simulink model "visualization"  (R2024a)
settings: Solver=VariableStepAuto  StartTime=0.0  StopTime=10.0  RelTol=1e-3
values from neighbouring files (symbols this model uses):
  enable_aircraft_view = 1    [main_chap05_02.m]
libraries: simulink x2
settings Model: Creator=pf  LastModifiedBy=pf

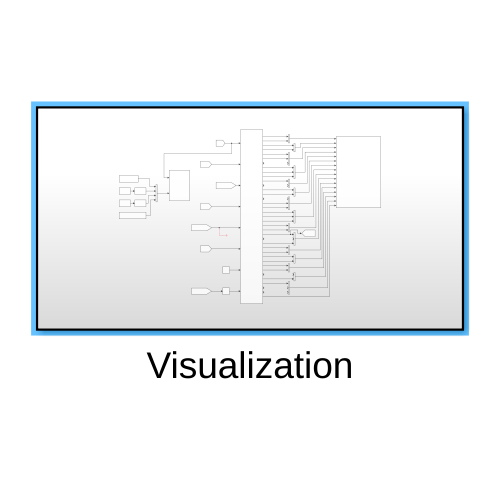
[thumbnail: Simulink's stored preview of the top-level diagram]
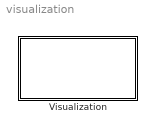
== system visualization ==
  Visualization : Subsystem

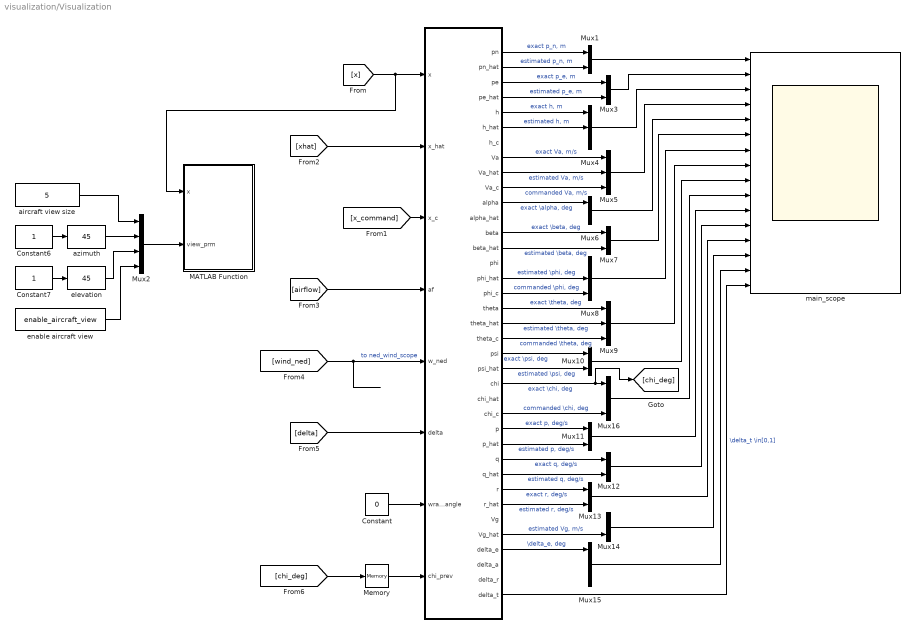
== system visualization/Visualization ==
  " " : MATLAB Function  TreatAsAtomicUnit=on
  Constant : Constant  Value=0
  Constant6 : Constant
  Constant7 : Constant
  MATLAB Function : MATLAB Function  TreatAsAtomicUnit=on
  Memory : Memory
  Mux{1,3,6..7,10..14} (9 alike) : Mux  Inputs=2
  Mux{4..5,8..9,15..16} (6 alike) : Mux  Inputs=3
  Mux2 : Mux
  aircraft view size : Constant  Value=5
  azimuth : simulink/Math Operations/Slider Gain  gain=45  low=-180  high=180
  elevation : simulink/Math Operations/Slider Gain  gain=45  low=-180  high=180
  enable aircraft view : Constant  Value=enable_aircraft_view
  main_scope : Scope  NumInputPorts=16
  wires:
  enable aircraft view/1 -> Mux2/4
  [x] -> MATLAB Function/1(x), " "/1(x)
  azimuth/1 -> Mux2/2
  Constant6/1 -> azimuth/1
  Constant7/1 -> elevation/1
  aircraft view size/1 -> Mux2/1
  Mux2/1 -> MATLAB Function/2(view_prm)
  elevation/1 -> Mux2/3
  [xhat] -> " "/2(x_hat)
  [x_command] -> " "/3(x_c)
  [airflow] -> " "/4(af)
  [wind_ned] -> " "/5(w_ned)  "to ned_wind_scope"
  [delta] -> " "/6(delta)
  Constant/1 -> " "/7(wrap_angle)
  " "/1(pn) -> Mux1/1  "exact p_n, m"
  " "/2(pn_hat) -> Mux1/2  "estimated p_n, m"
  " "/3(pe) -> Mux3/1  "exact p_e, m"
  " "/4(pe_hat) -> Mux3/2  "estimated p_e, m"
  " "/5(h) -> Mux4/1  "exact h, m"
  " "/6(h_hat) -> Mux4/2  "estimated h, m"
  " "/9(Va_hat) -> Mux5/2  "estimated Va, m/s"
  " "/10(Va_c) -> Mux5/3  "commanded Va, m/s"
  " "/8(Va) -> Mux5/1  "exact Va, m/s"
  " "/11(alpha) -> Mux6/1  "exact \\alpha, deg"
  " "/13(beta) -> Mux7/1  "exact \\beta, deg"
  " "/14(beta_hat) -> Mux7/2  "estimated \\beta, deg"
  " "/16(phi_hat) -> Mux8/2  "estimated \\phi, deg"
  " "/17(phi_c) -> Mux8/3  "commanded \\phi, deg"
  " "/19(theta_hat) -> Mux9/2  "estimated \\theta, deg"
  " "/18(theta) -> Mux9/1  "exact \\theta, deg"
  " "/20(theta_c) -> Mux9/3  "commanded \\theta, deg"
  " "/21(psi) -> Mux10/1  "exact \\psi, deg"
  " "/22(psi_hat) -> Mux10/2  "estimated \\psi, deg"
  " "/23(chi) -> [chi_deg], Mux16/1  "exact \\chi, deg"
  " "/25(chi_c) -> Mux16/3  "commanded \\chi, deg"
  " "/27(p_hat) -> Mux11/2  "estimated p, deg/s"
  " "/26(p) -> Mux11/1  "exact p, deg/s"
  " "/28(q) -> Mux12/1  "exact q, deg/s"
  " "/29(q_hat) -> Mux12/2  "estimated q, deg/s"
  " "/30(r) -> Mux13/1  "exact r, deg/s"
  " "/31(r_hat) -> Mux13/2  "estimated r, deg/s"
  " "/33(Vg_hat) -> Mux14/2  "estimated Vg, m/s"
  " "/34(delta_e) -> Mux15/1  "\\delta_e, deg"
  " "/37(delta_t) -> main_scope/16  "\\delta_t \\in[0,1]"
  Mux15/1 -> main_scope/15
  Mux14/1 -> main_scope/14
  Mux13/1 -> main_scope/13
  Mux12/1 -> main_scope/12
  Mux11/1 -> main_scope/11
  Mux9/1 -> main_scope/8
  Mux8/1 -> main_scope/7
  Mux7/1 -> main_scope/6
  Mux6/1 -> main_scope/5
  Mux5/1 -> main_scope/4
  Mux4/1 -> main_scope/3
  Mux3/1 -> main_scope/2
  Mux1/1 -> main_scope/1
  Mux10/1 -> main_scope/9
  Mux16/1 -> main_scope/10
  Memory/1 -> " "/8(chi_prev)
  [chi_deg] -> Memory/1

== matlab function visualization/Visualization/MATLAB Function ==
  data: x input; view_prm input
function draw_aircraft_fcn(x,view_prm)
    draw_aircraft(x,view_prm);
end

== matlab function visualization/Visualization/  ==
  data: x input; x_hat input; x_c input; af input; w_ned input; delta input; wrap_angle input; chi_prev input; pn output; pn_hat output; pe output; pe_hat output; h output; h_hat output; h_c output; Va output; Va_hat output; Va_c output; alpha output; alpha_hat output; beta output; beta_hat output; phi output; phi_hat output; phi_c output; theta output; theta_hat output; theta_c output; psi output; psi_hat output; chi output; chi_hat output; chi_c output; p output; p_hat output; q output; q_hat output; r output; r_hat output; Vg output; Vg_hat output; delta_e output; delta_a output; delta_r output; delta_t output
function [  pn, pn_hat, ...
            pe, pe_hat, ...
            h, h_hat, h_c, ...
            Va, Va_hat, Va_c, ...
            alpha, alpha_hat, ...
            beta, beta_hat, ...
            phi, phi_hat, phi_c, ...
            theta, theta_hat, theta_c, ...
            psi, psi_hat, ...
            chi, chi_hat, chi_c, ...
            p, p_hat, ...
            q, q_hat, ...
            r, r_hat, ...
            Vg, Vg_hat, ...
            delta_e,delta_a,delta_r,delta_t] = ...
            fcn(x,x_hat,x_c,af,w_ned,delta,wrap_angle,chi_prev)

    [  pn, pn_hat, ...
            pe, pe_hat, ...
            h, h_hat, h_c, ...
            Va, Va_hat, Va_c, ...
            alpha, alpha_hat, ...
            beta, beta_hat, ...
            phi, phi_hat, phi_c, ...
            theta, theta_hat, theta_c, ...
            psi, psi_hat, ...
            chi, chi_hat, chi_c, ...
            p, p_hat, ...
            q, q_hat, ...
            r, r_hat, ...
            Vg, Vg_hat, ...
            delta_e,delta_a,delta_r,delta_t] = ...
        xadec_postproc_ms(x,x_hat,x_c,af,w_ned,delta,wrap_angle,chi_prev);
end
